simulink model "sparse_parameter_test_simulink"  (R2016b)
settings: Solver=ode45  StartTime=0.0  StopTime=0.1  RelTol=1e-3
values from neighbouring files (symbols this model uses):
  input_update_port_first8 = ones(8*(N+1) + 1, 1)    [simulink_sparse_param_test.m]
  input_update_port_p12_stage3 = [1; 333]    [simulink_sparse_param_test.m]
  input_update_port_p12_stage6 = [0; 5000]    [simulink_sparse_param_test.m]
  input_update_port_p4243 = [1; 8*ones(2*(N+1), 1)]    [simulink_sparse_param_test.m]
settings Model: Creator=oj  LastModifiedBy=oj
settings DataIOCC: SaveFormat=StructureWithTime  ReturnWorkspaceOutputs=on
settings OptimizationCC: LifeSpan=inf
settings DebuggingCC: FcnCallInpInsideContextMsg=warning  SFExecutionAtInitializationDiag=none
settings HardwareCC: ProdBitPerSizeT=32  ProdBitPerPtrDiffT=32  ProdWordSize=32  ProdHWDeviceType=Specified
settings ModelReferenceCC: EnableRefExpFcnMdlSchedulingChecks=off
settings SFSimCC: SimUseLocalCustomCode=on
settings RTWCC: RTWUseLocalCustomCode=on

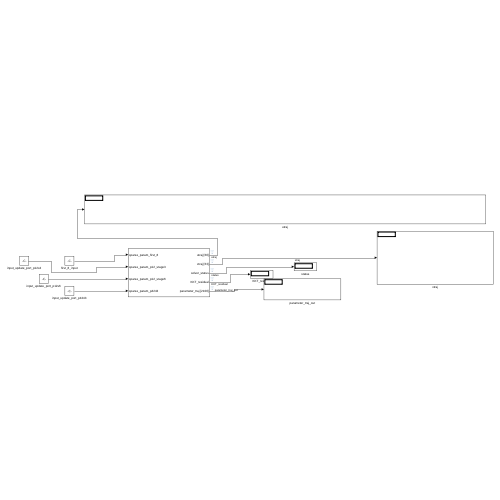
[thumbnail: Simulink's stored preview of the top-level diagram]
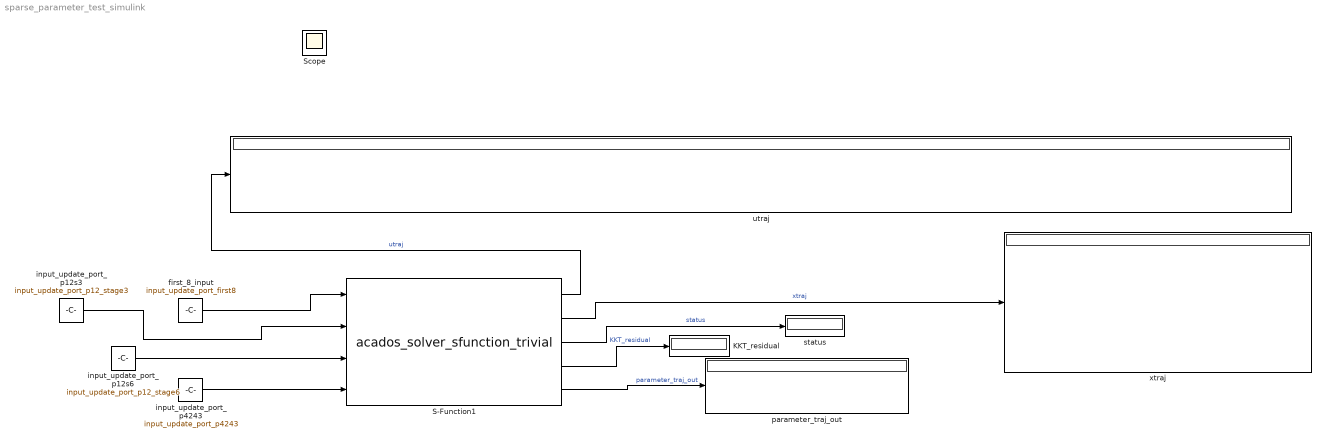
== system sparse_parameter_test_simulink ==
  KKT_residual : Display
  S-Function1 : S-Function  FunctionName=acados_solver_sfunction_trivial  SFunctionDeploymentMode=off  EnableBusSupport=off
      mask Display:
      | global sfun_input_names sfun_output_names
      | for i = 1:length(sfun_input_names)
      | 	port_label('input', i, sfun_input_names{i})
      | end
      | for i = 1:length(sfun_output_names)
      | 	port_label('output', i, sfun_output_names{i})
      | end
  first_8_input : Constant  Value=input_update_port_first8
  input_update_port_p12s3 : Constant  Value=input_update_port_p12_stage3
  input_update_port_p12s6 : Constant  Value=input_update_port_p12_stage6
  input_update_port_p4243 : Constant  Value=input_update_port_p4243
  parameter_traj_out : Display
  status : Display
  utraj : Display
  xtraj : Display
  Scope : Scope
  wires:
  S-Function1/3 -> status/1  "status"
  S-Function1/1 -> utraj/1  "utraj"
  S-Function1/2 -> xtraj/1  "xtraj"
  first_8_input/1 -> S-Function1/1
  S-Function1/5 -> parameter_traj_out/1  "parameter_traj_out"
  S-Function1/4 -> KKT_residual/1  "KKT_residual"
  input_update_port_p4243/1 -> S-Function1/4
  input_update_port_p12s6/1 -> S-Function1/3
  input_update_port_p12s3/1 -> S-Function1/2
